simulink subsystem "AirDragTorque"  (R2024b)
settings: Solver=VariableStepAuto  StartTime=0.0  StopTime=10.0  RelTol=1e-3
undefined symbols (not defined in the file): spacecraft
libraries: matrix_library x1, sadlib x1
settings Model: Creator=marco  LastModifiedBy=ferru

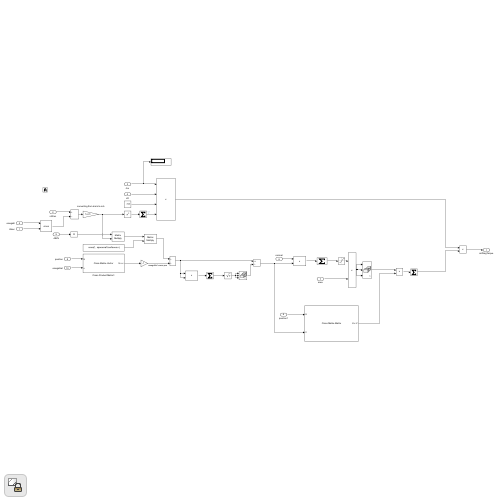
[thumbnail: Simulink's stored preview of the top-level diagram]
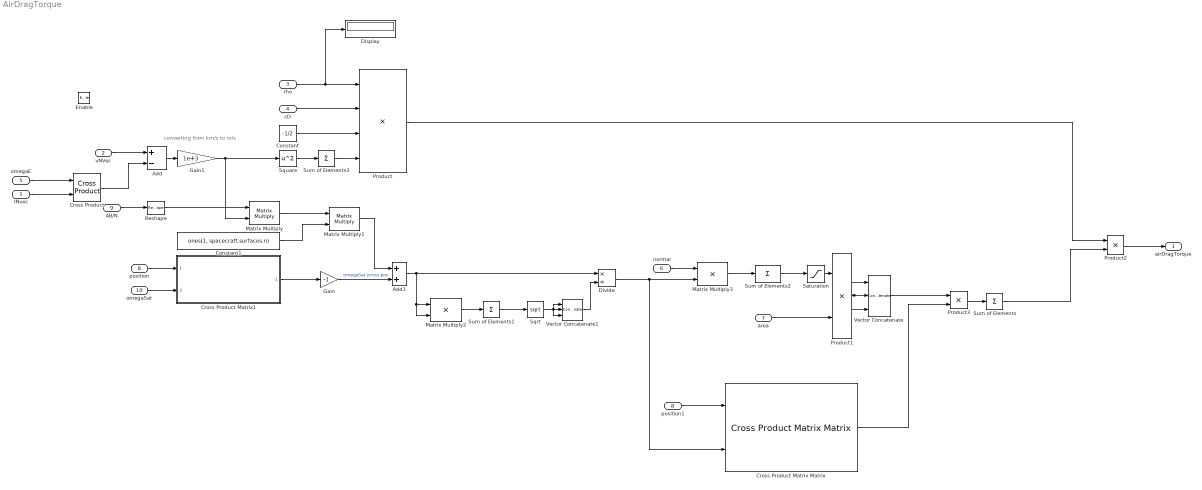
== system AirDragTorque ==
  note: converting from km/s to m/s
  rNvec : Inport
  vNVec : Inport  Port=2
  rho : Inport  Port=3
  cD : Inport  Port=4
  omegaE : Inport  Port=5
  normal : Inport  Port=6
  area : Inport  Port=7
  position : Inport  Port=8
  AB/N : Inport  Port=9
  omegaSat : Inport  Port=10
  Enable : EnablePort  StatesWhenEnabling=reset
  Add : Sum  Inputs=+-
  Add1 : Sum
  Constant : Constant  Value=-1/2
  Constant1 : Constant  Value=ones(1, spacecraft.surfaces.n)  VectorParams1D=off
  Cross Product : matrix_library/Cross Product
  Cross Product Matrix Matrix : sadlib/Cross Product Matrix Matrix
      settings: SourceProductName=SAD Library
  Cross Product Matrix1 : Subsystem  ReferencedSubsystem=CrossProductMatrix
  Display : Display
  Divide : Product  Inputs=*/
  Gain : Gain  Gain=-1
  Gain1 : Gain  Gain=1e+3
  Matrix Multiply : Product  Multiplication=Matrix(*)
  Matrix Multiply1 : Product  Multiplication=Matrix(*)
  Matrix Multiply2 : Product
  Matrix Multiply3 : Product
  Product : Product  Inputs=4
  Product1 : Product
  Product2 : Product
  Product3 : Product
  Reshape : Reshape  OutputDimensionality=Customize  OutputDimensions=[3, 3]
  Saturation : Saturate  UpperLimit=inf  LowerLimit=0
  Sqrt : Sqrt
  Square : Math  Operator=square
  Sum of Elements : Sum  Inputs=+  CollapseMode=Specified dimension  CollapseDim=2
  Sum of Elements1 : Sum  Inputs=+  CollapseMode=Specified dimension
  Sum of Elements2 : Sum  Inputs=+  CollapseMode=Specified dimension
  Sum of Elements3 : Sum  Inputs=+
  Vector Concatenate : Concatenate  NumInputs=3  Mode=Multidimensional array
  Vector Concatenate1 : Concatenate  NumInputs=3  Mode=Multidimensional array
  position1 : InportShadow  Port=8
  airDragTorque : Outport
  wires:
  Add/1 -> Gain1/1
  Cross Product Matrix Matrix/1 -> Product3/2
  position1/1 -> Cross Product Matrix Matrix/1
  Gain/1 -> Add1/2  "omegaSat \\cross pos"
  Sqrt/1 -> Vector Concatenate1/3, Vector Concatenate1/1, Vector Concatenate1/2
  Sum of Elements2/1 -> Saturation/1
  Vector Concatenate1/1 -> Divide/2
  Sum of Elements1/1 -> Sqrt/1
  Matrix Multiply2/1 -> Sum of Elements1/1
  Matrix Multiply1/1 -> Add1/1
  Constant1/1 -> Matrix Multiply1/2
  Matrix Multiply/1 -> Matrix Multiply1/1
  normal/1 -> Matrix Multiply3/1
  Vector Concatenate/1 -> Product3/1
  Product1/1 -> Vector Concatenate/2, Vector Concatenate/3, Vector Concatenate/1
  Sum of Elements/1 -> Product2/2
  Product3/1 -> Sum of Elements/1
  Product2/1 -> airDragTorque/1
  Product/1 -> Product2/1
  Divide/1 -> Matrix Multiply3/2, Cross Product Matrix Matrix/2
  area/1 -> Product1/2
  Matrix Multiply3/1 -> Sum of Elements2/1
  Add1/1 -> Matrix Multiply2/2, Matrix Multiply2/1, Divide/1
  Cross Product Matrix1/1 -> Gain/1
  position/1 -> Cross Product Matrix1/1
  omegaSat/1 -> Cross Product Matrix1/2
  Reshape/1 -> Matrix Multiply/1
  AB/N/1 -> Reshape/1
  rho/1 -> Product/1, Display/1
  cD/1 -> Product/2
  Constant/1 -> Product/3
  Square/1 -> Sum of Elements3/1
  Gain1/1 -> Matrix Multiply/2, Square/1
  Cross Product/1 -> Add/2
  vNVec/1 -> Add/1
  rNvec/1 -> Cross Product/2
  omegaE/1 -> Cross Product/1
  Sum of Elements3/1 -> Product/4
  Saturation/1 -> Product1/1
